simulink model "L9_sim"  (R2022b)
settings: Solver=VariableStepAuto  StartTime=0.0  StopTime=20  RelTol=1e-3
undefined symbols (not defined in the file): dem_cn, num_cn, T, Ts
settings Model: Creator=xinz  LastModifiedBy=xinz

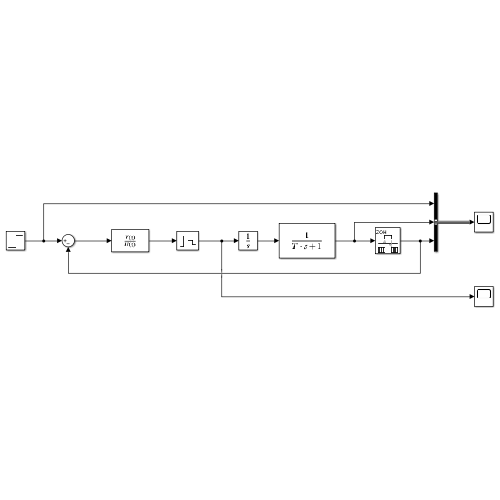
[thumbnail: Simulink's stored preview of the top-level diagram]
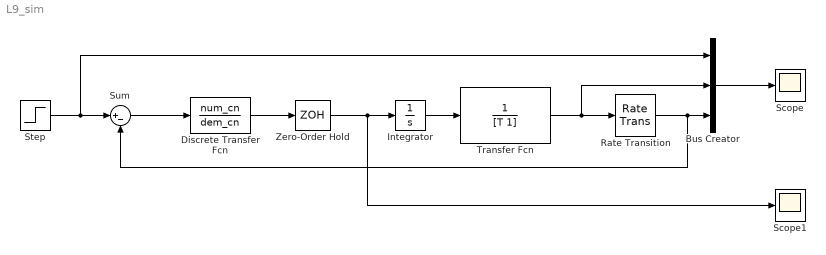
== system L9_sim ==
  Bus Creator : BusCreator  Inputs=3
  Discrete Transfer Fcn : DiscreteTransferFcn  Numerator=num_cn  Denominator=dem_cn  SampleTime=Ts
  Integrator : Integrator
  Rate Transition : RateTransition  OutPortSampleTime=Ts
  Scope : Scope
  Scope1 : Scope
  Step : Step  SampleTime=0
  Sum : Sum  Inputs=|+-
  Transfer Fcn : TransferFcn  Denominator=[T 1]
  Zero-Order Hold : ZeroOrderHold  SampleTime=Ts
  wires:
  Integrator/1 -> Transfer Fcn/1
  Sum/1 -> Discrete Transfer Fcn/1
  Discrete Transfer Fcn/1 -> Zero-Order Hold/1
  Zero-Order Hold/1 -> Scope1/1, Integrator/1
  Rate Transition/1 -> Sum/2, Bus Creator/3
  Transfer Fcn/1 -> Bus Creator/2, Rate Transition/1
  Step/1 -> Bus Creator/1, Sum/1
  Bus Creator/1 -> Scope/1
